simulink model "furuta_pi_hardware_verify"  (R2026b)
settings: Solver=FixedStepDiscrete  StopTime=inf  FixedStep=0.005  EnableMultiTasking=on
model workspace (MAT data in the model file):
  calibration = [-209.05 -1 4058.5 1]
  drive = [0 0 0 0]
  limits = [0 0 0 0]
libraries: raspberrypiCommlib x4
settings Model: Creator=Lsh  LastModifiedBy=Lsh
settings SolverCC: PositivePriorityOrder=on
settings OptimizationCC: DifferentSizesBufferReuse=on  EfficientTunableParamExpr=on  EnhancedBackFolding=on  MaxStackSize=200000  OptimizationCustomize=off  OptimizeBlockOrder=speed  PassReuseOutputArgsAs=Individual arguments  RemoveInternalMemoryZeroInit=on  RemoveRootLevelIOMemoryZeroInit=on
settings DebuggingCC: ParameterTunabilityLossMsg=error
settings HardwareCC: ProdHWDeviceType=ARM Compatible->ARM Cortex-A (64-bit)  ProdLargestAtomicFloat=Double  ProdLargestAtomicInteger=LongLong  ProdLongLongMode=on
settings RTWCC: BuildConfiguration=Faster Runs  Description=Embedded Coder  HardwareBoard=Raspberry Pi (64bit)  SystemTargetFile=ert.tlc  TLCOptions="-aInlineSetEventsForThisBaseRateFcn=TLC_FALSE -aSuppressMultiTaskScheduler=TLC_FALSE  -aRateBasedStepFcn=0"  TemplateMakefile=ert_default_tmf  Toolchain=GNU GCC RPIUtils
settings CodeAppCC: ForceParamTrailComments=on  IgnoreCustomStorageClasses=off  InsertBlockDesc=on  OperatorAnnotations=on  SFDataObjDesc=on  SimulinkDataObjDesc=on
settings ERTTargetCC: CombineSignalStateStructs=on  ExtModeIntrfLevel=Level2 - Open  ExtModeMexFile=ext_xcp  ExtModeStaticAlloc=on  SupportVariableSizeSignals=on

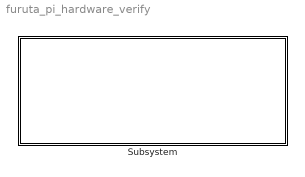
== system furuta_pi_hardware_verify ==
  Subsystem : Subsystem

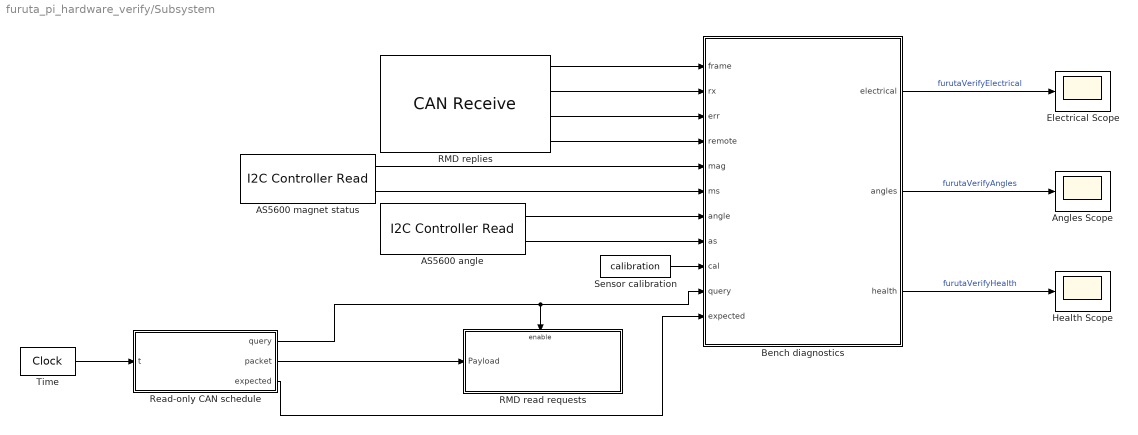
== system furuta_pi_hardware_verify/Subsystem ==
  AS5600 angle : raspberrypiCommlib/I2C Controller Read  BoardProperty=Pi 5 Model  I2CModule=1  Mode=Master  SlaveAddress=54  SlaveByteOrder=BigEndian  Direction=Receiver  RegisterAddressMode=on  RegisterAddress=14  SlaveDataType=uint8  DataLength=2  NoAck=off  RepeatedStart=on  OutputStatus=on  SampleTime=.005
  AS5600 magnet status : raspberrypiCommlib/I2C Controller Read  BoardProperty=Pi 5 Model  I2CModule=1  Mode=Master  SlaveAddress=54  SlaveByteOrder=BigEndian  Direction=Receiver  RegisterAddressMode=on  RegisterAddress=11  SlaveDataType=uint8  DataLength=1  NoAck=off  RepeatedStart=on  OutputStatus=on  SampleTime=.005
  Angles Scope : Scope
      settings: ActiveDisplayYMinimum=-455.4093776239414  ActiveDisplayYMaximum=2333.4517063604335
  Bench diagnostics : MATLAB Function  TreatAsAtomicUnit=on
  Electrical Scope : Scope
      settings: ActiveDisplayYMinimum=-0.25827039430690535  ActiveDisplayYMaximum=0.21229722748795721
  Health Scope : Scope
      settings: ActiveDisplayYMinimum=-12.867521604726848  ActiveDisplayYMaximum=12.6581096452732
  RMD read requests : Subsystem  TreatAsAtomicUnit=on
  RMD replies : raspberrypiCommlib/CAN Receive  DeviceID=can0  SetupCAN=off  TypeofCAN=Real  OutputDataType=Raw data  IdentifierType=Standard (11-bit identifier)  MessageId=577  MsgLength=8  SampleTime=.005  OutputError=on  OutputRemote=on  SimulateUsing=Code generation
  Read-only CAN schedule : MATLAB Function  TreatAsAtomicUnit=on
  Sensor calibration : Constant  Value=calibration  SampleTime=.005
  Time : DigitalClock  SampleTime=.005
  wires:
  AS5600 magnet status/2 -> Bench diagnostics/6(ms)
  RMD replies/4 -> Bench diagnostics/4(remote)
  RMD replies/1 -> Bench diagnostics/1(frame)
  AS5600 magnet status/1 -> Bench diagnostics/5(mag)
  Read-only CAN schedule/2(packet) -> RMD read requests/1(Payload)
  RMD replies/2 -> Bench diagnostics/2(rx)
  Bench diagnostics/1(electrical) -> Electrical Scope/1  "furutaVerifyElectrical"
  RMD replies/3 -> Bench diagnostics/3(err)
  Bench diagnostics/2(angles) -> Angles Scope/1  "furutaVerifyAngles"
  AS5600 angle/1 -> Bench diagnostics/7(angle)
  AS5600 angle/2 -> Bench diagnostics/8(as)
  Sensor calibration/1 -> Bench diagnostics/9(cal)
  Bench diagnostics/3(health) -> Health Scope/1  "furutaVerifyHealth"
  Read-only CAN schedule/1(query) -> RMD read requests/Enable, Bench diagnostics/10(query)
  Time/1 -> Read-only CAN schedule/1(t)
  Read-only CAN schedule/3(expected) -> Bench diagnostics/11(expected)

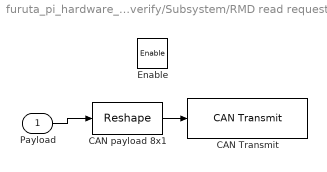
== system furuta_pi_hardware_verify/Subsystem/RMD read requests ==
  Payload : Inport
  Enable : EnablePort
  CAN Transmit : raspberrypiCommlib/CAN Transmit  DeviceID=can0  SetupCAN=off  TypeofCAN=Real  InputDataType=Raw data  BlockingMode_=off  BlockTimeout_=1  OutputStatus=off  IdentifierType=Standard (11-bit identifier)  MessageId=321  MsgLength=8  RemoteFrame=off  SimulateUsing=Code generation
  CAN payload 8x1 : Reshape  OutputDimensionality=Customize  OutputDimensions=[8 1]
  wires:
  Payload/1 -> CAN payload 8x1/1
  CAN payload 8x1/1 -> CAN Transmit/1

== matlab function furuta_pi_hardware_verify/Subsystem/Bench diagnostics ==
  data: frame input; electrical output; rx input; err input; remote input; mag input; ms input; angle input; as input; cal input; query input; expected input; angles output; health output
function [electrical,angles,health] = diagnostics(frame,rx,err,remote,mag,ms,angle,as,cal,query,expected)
[electrical,angles,health] = furuta_pi_verify_sample(frame,rx,err,remote,mag,ms,angle,as,cal,query,expected);
end

== matlab function furuta_pi_hardware_verify/Subsystem/Read-only CAN schedule ==
  data: query output; t input; packet output; expected output
function [query,packet,expected] = schedule(t)
tick = round(t/.005);
codes = uint8([146 154 156]);
expected = codes(mod(floor(tick/2),3)+1);
query = mod(tick,2)==0;
packet = [expected zeros(1,7,'uint8')];
end
